simulink model "test_SimulinkMdl4_Baseline"  (R2021b)
settings: Solver=FixedStepAuto  StartTime=0.0  StopTime=400  FixedStep=DT  RelTol=1e-3
PreLoadFcn:
  | % dataInPath = fullfile(fileparts(pwd),'dataIn');
  | % addpath(dataInPath);
  | % addpath(fullfile(pwd,'dataOut'));
  | % addpath(genpath('C:\Projects\FASTTool'));
  | % addpath('subfunctionsMPC')
  | % addpath('MDlWECS')
  | % onlyInit = 1;
  | % dataInPath = fullfile(fileparts(pwd),'dataIn');
  | % load(fullfile(dataInPath,'OutDataSweep.mat'),'OutTable'); %#ok<NASGU>
  | % DT = 0.008;
values from neighbouring files (symbols this model uses):
  DT = 0.008    [dataDLR.m]    (also in generateReport.m; initLPVParam.m; initWorkspace.m; runCalculateEvalCriteria.m)
  Lin_points : value not decoded    [DD_test.sldd]
undefined symbols (not defined in the file or in its folder): Rotor_Lambda
settings Model: DataDictionary=DD_test.sldd  Creator=Hazim Namik  LastModifiedBy=ditt_aj
settings SolverCC: AlgebraicLoopSolver=TrustRegion
settings DataIOCC: LimitDataPoints=on  SaveFormat=Array  ReturnWorkspaceOutputs=off
settings OptimizationCC: BlockReduction=off  BooleanDataType=off  LifeSpan=inf
settings DebuggingCC: SaveWithParameterizedLinksMsg=none  UnderspecifiedInitializationDetection=Classic  MergeDetectMultiDrivingBlocksExec=none  SignalResolutionControl=TryResolveAllWithWarning  SFUnexpectedBacktrackingDiag=warning  SFNoUnconditionalDefaultTransitionDiag=warning  SFExecutionAtInitializationDiag=none  SFMachineParentedDataDiag=warning  ArithmeticOperatorsInVariantConditions=warning
settings HardwareCC: ProdBitPerPointer=32  ProdBitPerSizeT=32  ProdBitPerPtrDiffT=32  ProdLargestAtomicFloat=None  ProdIntDivRoundTo=Undefined  ProdEndianess=Unspecified  ProdWordSize=32  ProdHWDeviceType=32-bit Generic  TargetUnknown=on
settings ModelReferenceCC: PropagateSignalLabelsOutOfModel=off
settings SFSimCC: SimUseLocalCustomCode=off  CustomCodeUndefinedFunction=UseInterfaceOnly
settings RTWCC: RTWUseLocalCustomCode=off
settings CodeAppCC: StateflowObjectComments=on
settings GRTTargetCC: TargetLangStandard=C89/C90 (ANSI)
settings ConfigComp: CovMetricSettings=dw  CovSaveCumulativeToWorkspaceVar=on  CovSaveSingleToWorkspaceVar=on  CovExternalEMLEnable=off

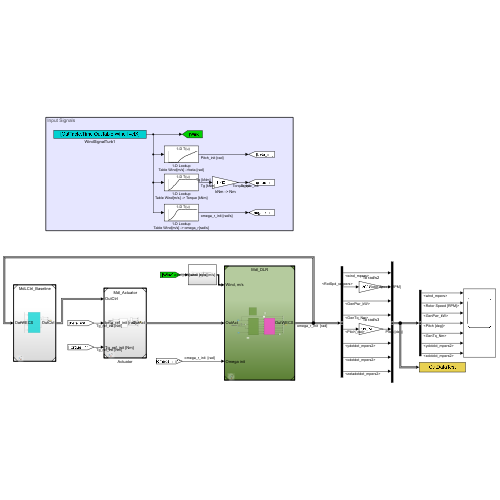
[thumbnail: Simulink's stored preview of the top-level diagram]
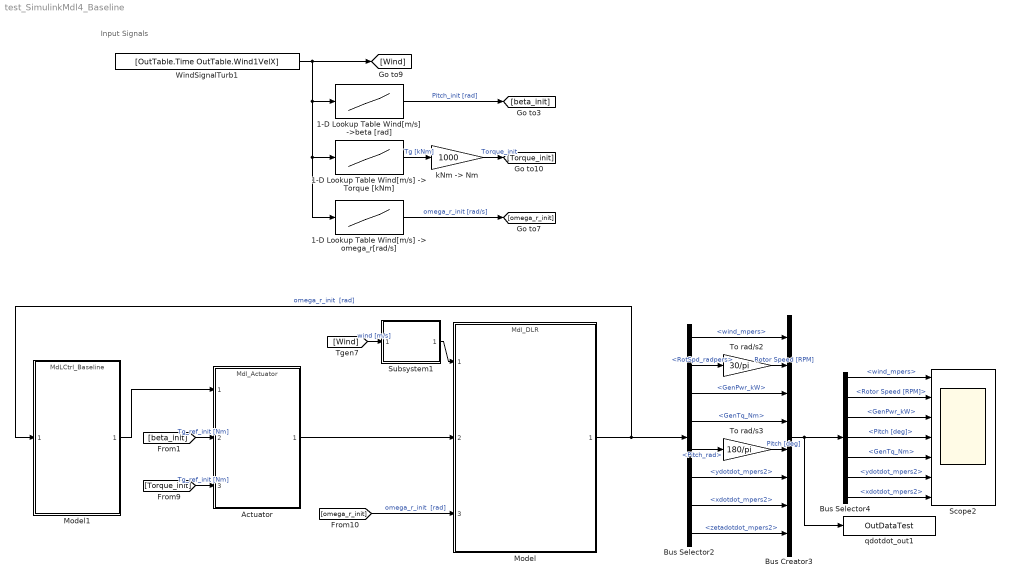
== system test_SimulinkMdl4_Baseline ==
  note: Input Signals
  "1-D Lookup Table Wind[m/s] -> Torque [kNm]" : Lookup_n-D  NumberOfTableDimensions=1  BreakpointsForDimension1=Lin_points.V  BreakpointsForDimension2=Rotor_Lambda  Table=Lin_points.Torque  InternalRulePriority=Speed  RndMeth=Simplest  InputSameDT=on
  "1-D Lookup Table Wind[m/s] -> omega_r[rad/s]" : Lookup_n-D  NumberOfTableDimensions=1  BreakpointsForDimension1=Lin_points.V  BreakpointsForDimension2=Rotor_Lambda  Table=Lin_points.RSpeed  InternalRulePriority=Speed  RndMeth=Simplest  InputSameDT=on
  1-D Lookup Table Wind[m/s] ->beta [rad] : Lookup_n-D  NumberOfTableDimensions=1  BreakpointsForDimension1=Lin_points.V  BreakpointsForDimension2=Rotor_Lambda  Table=Lin_points.Pitch  InternalRulePriority=Speed  RndMeth=Simplest  InputSameDT=on
  Actuator : ModelReference  ModelNameDialog=Mdl_Actuator.slx  SimulationMode=Normal  ModelReferenceVersion=1.18
  Bus Creator3 : BusCreator  Inputs=8
  Bus Selector2 : BusSelector  OutputSignals=wind_mpers,RotSpd_radpers,GenPwr_kW,GenTq_Nm,Pitch_rad,ydotdot_mpers2,xdotdot_mpers2,zetadotdot_mpers2
  Bus Selector4 : BusSelector  OutputSignals=wind_mpers,Rotor Speed [RPM],GenPwr_kW,Pitch [deg],GenTq_Nm,ydotdot_mpers2,xdotdot_mpers2
  Model : ModelReference  ModelNameDialog=Mdl_DLR.mdl  SimulationMode=Normal  ModelReferenceVersion=5.2
  Model1 : ModelReference  ModelNameDialog=MdLCtrl_Baseline.slx  SimulationMode=Normal  ModelReferenceVersion=4.1
  Scope2 : Scope  NumInputPorts=7
      settings: Tag=Scope
  Subsystem1 : Subsystem
  To rad/s2 : Gain  Gain=30/pi
  To rad/s3 : Gain  Gain=180/pi
  WindSignalTurb1 : FromWorkspace  VariableName=[OutTable.Time OutTable.Wind1VelX]  SampleTime=DT  OutputAfterFinalValue=Holding final value
  "kNm -> Nm" : Gain  Gain=1000
  qdotdot_out1 : ToWorkspace  VariableName=OutDataTest  SampleTime=-1
  wires:
  [omega_r_init] -> Model/3  "omega_r_init  [rad]"
  [Wind] -> Subsystem1/1(wind  [m/s])  "wind [m/s]"
  "1-D Lookup Table Wind[m/s] -> Torque [kNm]"/1 -> "kNm -> Nm"/1  "Tg [kNm]"
  WindSignalTurb1/1 -> [Wind], "1-D Lookup Table Wind[m/s] -> omega_r[rad/s]"/1, "1-D Lookup Table Wind[m/s] -> Torque [kNm]"/1, 1-D Lookup Table Wind[m/s] ->beta [rad]/1
  Actuator/1 -> Model/2
  Subsystem1/1(wind x,y,z [m/s]) -> Model/1
  [Torque_init] -> Actuator/3  "Tg_ref_init [Nm]"
  "1-D Lookup Table Wind[m/s] -> omega_r[rad/s]"/1 -> [omega_r_init]  "omega_r_init [rad/s]"
  "kNm -> Nm"/1 -> [Torque_init]  "Torque_init"
  1-D Lookup Table Wind[m/s] ->beta [rad]/1 -> [beta_init]  "Pitch_init [rad]"
  Model1/1 -> Actuator/1
  [beta_init] -> Actuator/2  "Tg_ref_init [Nm]"
  Bus Selector2/2 -> To rad/s2/1  "<RotSpd_radpers>"
  Bus Selector4/1 -> Scope2/1  "<wind_mpers>"
  Bus Selector4/6 -> Scope2/6  "<ydotdot_mpers2>"
  To rad/s3/1 -> Bus Creator3/5  "Pitch [deg]"
  Bus Selector4/4 -> Scope2/4  "<Pitch [deg]>"
  Bus Selector2/1 -> Bus Creator3/1  "<wind_mpers>"
  To rad/s2/1 -> Bus Creator3/2  "Rotor Speed [RPM]"
  Bus Selector4/2 -> Scope2/2  "<Rotor Speed [RPM]>"
  Bus Selector2/8 -> Bus Creator3/8  "<zetadotdot_mpers2>"
  Bus Selector2/4 -> Bus Creator3/4  "<GenTq_Nm>"
  Bus Creator3/1 -> Bus Selector4/1, qdotdot_out1/1
  Bus Selector4/5 -> Scope2/5  "<GenTq_Nm>"
  Bus Selector2/3 -> Bus Creator3/3  "<GenPwr_kW>"
  Bus Selector4/7 -> Scope2/7  "<xdotdot_mpers2>"
  Bus Selector2/6 -> Bus Creator3/6  "<ydotdot_mpers2>"
  Model/1 -> Model1/1, Bus Selector2/1  "omega_r_init  [rad]"
  Bus Selector2/5 -> To rad/s3/1  "<Pitch_rad>"
  Bus Selector2/7 -> Bus Creator3/7  "<xdotdot_mpers2>"
  Bus Selector4/3 -> Scope2/3  "<GenPwr_kW>"

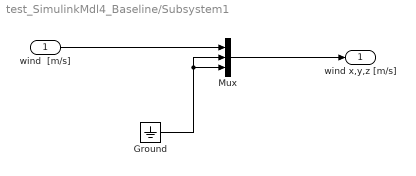
== system test_SimulinkMdl4_Baseline/Subsystem1 ==
  wind  [m/s] : Inport
  Ground : Ground
  Mux : Mux  Inputs=3
  wind x,y,z [m/s] : Outport
  wires:
  wind  [m/s]/1 -> Mux/1
  Mux/1 -> wind x,y,z [m/s]/1
  Ground/1 -> Mux/3, Mux/2
